simulink model "asbCubeSatVisualization"  (R2025b)
settings: configuration reference "CubeSatConfigSet" (kept outside this file)
StopFcn:
  | exSatScenMdl = bdroot(gcs);
  | exSatScenBlk = exSatScenMdl + "/Satellite Scenario Playback";
  | 
  | % If workspace blocks are stored in single output variable, need to access from there
  | if get_param(exSatScenMdl, "ReturnWorkspaceOutputs") == "on"
  |     exSatScenOutVar = get_param(exSatScenMdl, "ReturnWorkspaceOutputsName");
  |     if exist(exSatScenOutVar, "var")
  |         exSatScenTimeData = eval(exSatScenOutVar).exSatScenTimeData;
  |         exSatScenPositionData = eval(exSatScenOutVar).exSatScenPositionData;
  |         exSatScenVelocityData = eval(exSatScenOutVar).exSatScenVelocityData;
  |         exSatScenAttitudeData = eval(exSatScenOutVar).exSatScenAttitudeData;
  |     end
  | end
  | 
  | % If variables exist, create scenario (variables are not created if called with sim command)
  | if exist("exSatScenTimeData", "var") && exist("exSatScenPositionData", "var") && exist("exSatScenVelocityData", "var") && exist("exSatScenAttitudeData", "var")
  |     % Create satellite scenario from variables accessed above or directly from workspace
  |     exSatScenario = Aero.spacecraft.analysis.createSatelliteScenarioFromSim(exSatScenBlk, ...
  |         exSatScenTimeData, exSatScenPositionData, exSatScenVelocityData, exSatScenAttitudeData);
  | end
  | 
  | clear exSatScenBlk exSatScenMdl exSatScenOutVar exSatScenTimeData exSatScenPositionData exSatScenVelocityData exSatScenAttitudeData
libraries: simulink x12
settings Model: DataDictionary=asbCubeSatArchInterfaceData.sldd  Creator=The MathWorks, Inc.  LastModifiedBy=The MathWorks, Inc.
settings ConfigSetRef: SourceName=CubeSatConfigSet

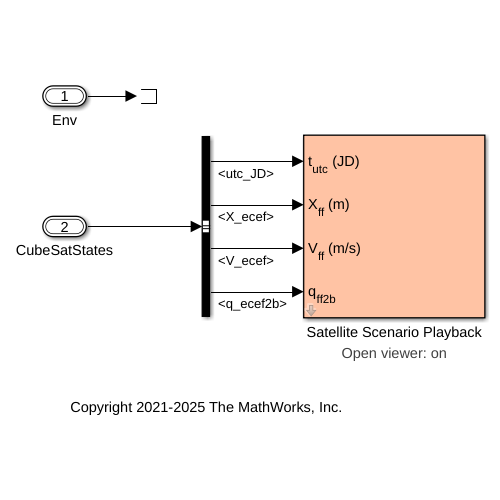
[thumbnail: Simulink's stored preview of the top-level diagram]
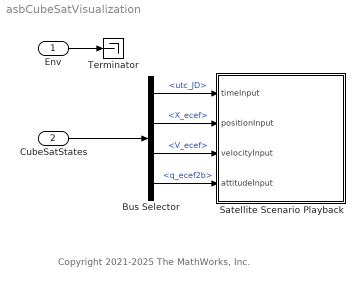
== system asbCubeSatVisualization ==
  note: Copyright 2021-2025 The MathWorks, Inc.
  Env : Inport  OutDataTypeStr=Bus: EnvBus
  CubeSatStates : Inport  Port=2  OutDataTypeStr=Bus: StatesOutBus
  Bus Selector : BusSelector  OutputSignals=utc_JD,X_ecef,V_ecef,q_ecef2b
  Satellite Scenario Playback : Subsystem  mask{openViewer=on, stateFrame=ECEF (Fixed-frame), useVelocity=on, useAttitude=on, attitudeFrame=ECEF (Fixed-frame), satName=Satellite, showTriad=on, show3dModel=on, showFOV=on, fovHalfAngle=30, scenarioStep=60}
      mask prompts: openViewer "Enable Satellite Scenario Viewer playback animation"; stateFrame "State coordinate frame:"; useVelocity "Add velocity port"; useAttitude "Add attitude port"; attitudeFrame "Attitude coordinate frame (Frame to Body):"; satName "Satellite or constellation label:"; showTriad "Show coordinate axis triad (Body frame)"; show3dModel "Show 3D satellite model"; showFOV "Add sensor field-of-view (FOV)"; fovHalfAngle "FOV half angle (deg):"; scenarioStep "Satellite scenario sample time (s):"
      mask init:
      | ports = Aero.spacecraft.analysis.satelliteScenarioPlaybackMaskCallback(gcb, "init");
      settings: AttributesFormatString=Open viewer: %<openViewer>
      mask Callback openViewer: Aero.spacecraft.analysis.satelliteScenarioPlaybackMaskCallback(gcb, "viewer");
      mask TypeOptions stateFrame: Inertial (ICRF) | ECEF (Fixed-frame) | Geographic
      mask Callback useAttitude: Aero.spacecraft.analysis.satelliteScenarioPlaybackMaskCallback(gcb, "attitude");
      mask TypeOptions attitudeFrame: Inertial (ICRF) | ECEF (Fixed-frame) | NED
      mask Callback showFOV: Aero.spacecraft.analysis.satelliteScenarioPlaybackMaskCallback(gcb, "fov");
      mask DialogControl DescGroupVar Prompt: Satellite Scenario Viewer Playback Animation
      mask DialogControl DescTextVar Prompt: <html><p>Create a satellite scenario object and launch the Satellite Scenario Viewer using the trajectories provided as inputs to the block.</p><p>If playback animation is enabled, the block opens Satellite Scenario Viewer after the model simulation has stopped. The viewer will not launch if the model is run using the <tt>sim</tt> command.</p> <p>To add additional satellites, ground stations, or platforms to the scenario and perform mission analysis, including line-of-sight access and eclipse analysis, use the base workspace variable <tt>exSatScenario</tt>.</p></html>
      mask DialogControl Container3 Prompt: Parameters
      mask DialogControl Container4 Prompt: Trajectory
      mask DialogControl ParameterGroupVar Prompt: Playback
      mask DialogControl SatelliteScenarioPlaybackTag Prompt: SatelliteScenarioPlaybackTag
      mask Display:
      | port_label(ports(1).type,ports(1).port,ports(1).txt,'texmode','on');
      | port_label(ports(2).type,ports(2).port,ports(2).txt,'texmode','on');
      | port_label(ports(3).type,ports(3).port,ports(3).txt,'texmode','on');
      | port_label(ports(4).type,ports(4).port,ports(4).txt,'texmode','on');
  Terminator : Terminator
  wires:
  CubeSatStates/1 -> Bus Selector/1
  Env/1 -> Terminator/1
  Bus Selector/4 -> Satellite Scenario Playback/4(attitudeInput)  "<q_ecef2b>"
  Bus Selector/3 -> Satellite Scenario Playback/3(velocityInput)  "<V_ecef>"
  Bus Selector/2 -> Satellite Scenario Playback/2(positionInput)  "<X_ecef>"
  Bus Selector/1 -> Satellite Scenario Playback/1(timeInput)  "<utc_JD>"

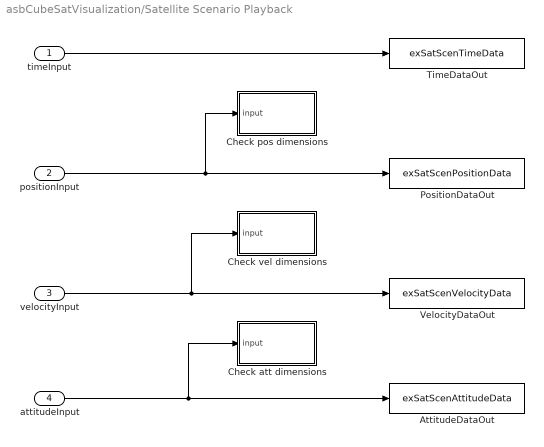
== system asbCubeSatVisualization/Satellite Scenario Playback ==
  timeInput : Inport  PortDimensions=1
  positionInput : Inport  Port=2  Unit=m
  velocityInput : Inport  Port=3  Unit=m/s
  attitudeInput : Inport  Port=4
  AttitudeDataOut : ToWorkspace  VariableName=exSatScenAttitudeData  SampleTime=-1
  Check att dimensions : Subsystem  mask{N=4, AssertionFailFcn=error("Attitude input must be be a vector with 4 elements or a 2-D array of size [m x 4].")}
      mask prompts: N "State dimension (N):"; AssertionFailFcn "Simulink:blkprm_prompts:AssertionCallback"
      mask TypeOptions AssertionFailFcn: Assertion/AssertionFailFcn | Second check/Assertion/AssertionFailFcn
      mask DialogControl DescGroupVar Prompt: Assert expected dimensions
      mask DialogControl DescTextVar Prompt: Assert that input signal is size N or size M x N where M is the number of satellites. N is 3 for position and velocity, and 4 for attitude (quaternions).
      mask DialogControl AssertionFailFcn Prompt: Simulation callback when assertion fails:
  Check pos dimensions : Subsystem  mask{N=3, AssertionFailFcn=error("Position input must be be a vector with 3 elements or a 2-D array of size [m x 3].")}
      mask prompts: N "State dimension (N):"; AssertionFailFcn "Simulink:blkprm_prompts:AssertionCallback"
      mask TypeOptions AssertionFailFcn: Assertion/AssertionFailFcn | Second check/Assertion/AssertionFailFcn
      mask DialogControl DescGroupVar Prompt: Assert expected dimensions
      mask DialogControl DescTextVar Prompt: Assert that input signal is size N or size M x N where M is the number of satellites. N is 3 for position and velocity, and 4 for attitude (quaternions).
      mask DialogControl AssertionFailFcn Prompt: Simulation callback when assertion fails:
  Check vel dimensions : Subsystem  mask{N=3, AssertionFailFcn=error("Velocity input must be be a vector with 3 elements or a 2-D array of size [m x 3].")}
      mask prompts: N "State dimension (N):"; AssertionFailFcn "Simulink:blkprm_prompts:AssertionCallback"
      mask TypeOptions AssertionFailFcn: Assertion/AssertionFailFcn | Second check/Assertion/AssertionFailFcn
      mask DialogControl DescGroupVar Prompt: Assert expected dimensions
      mask DialogControl DescTextVar Prompt: Assert that input signal is size N or size M x N where M is the number of satellites. N is 3 for position and velocity, and 4 for attitude (quaternions).
      mask DialogControl AssertionFailFcn Prompt: Simulation callback when assertion fails:
  PositionDataOut : ToWorkspace  VariableName=exSatScenPositionData  SampleTime=-1
  TimeDataOut : ToWorkspace  VariableName=exSatScenTimeData  SampleTime=-1
  VelocityDataOut : ToWorkspace  VariableName=exSatScenVelocityData  SampleTime=-1
  wires:
  positionInput/1 -> PositionDataOut/1, Check pos dimensions/1(input)
  velocityInput/1 -> Check vel dimensions/1(input), VelocityDataOut/1
  attitudeInput/1 -> Check att dimensions/1(input), AttitudeDataOut/1
  timeInput/1 -> TimeDataOut/1

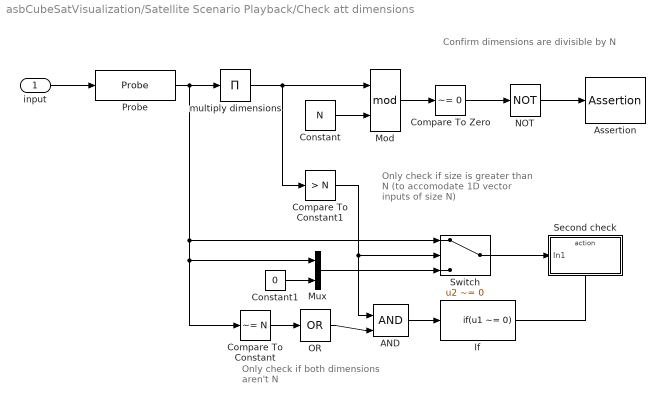
== system asbCubeSatVisualization/Satellite Scenario Playback/Check att dimensions ==
  note: Only check if both dimensions aren't N
  note: Only check if size is greater than N (to accomodate 1D vector inputs of size N)
  note: Confirm dimensions are divisible by N
  input : Inport
  AND : Logic  IconShape=distinctive  AllPortsSameDT=off  OutDataTypeStr=boolean
  Assertion : Assertion  AssertionFailFcn="error(\"Attitude input must be be a vector with 4 elements or a 2-D array of size [m x 4].\")"
  Compare To Constant : simulink/Logic and Bit Operations/Compare To Constant  relop=~=  const=N  OutDataTypeStr=boolean  ZeroCross=off
  Compare To Constant1 : simulink/Logic and Bit Operations/Compare To Constant  relop=>  const=N  OutDataTypeStr=boolean  ZeroCross=off
  Compare To Zero : simulink/Logic and Bit Operations/Compare To Zero  relop=~=  OutDataTypeStr=boolean  ZeroCross=off
  Constant : Constant  Value=N  OutDataTypeStr=uint8
  Constant1 : Constant  Value=0  OutDataTypeStr=uint8
  If : If  IfExpression=u1 ~= 0  ShowElse=off  ZeroCross=off
  Mod : Math  Operator=mod
  Mux : Mux  Inputs=2
  NOT : Logic  Operator=NOT  IconShape=distinctive  AllPortsSameDT=off  OutDataTypeStr=boolean
  OR : Logic  Operator=OR  Inputs=1  IconShape=distinctive  AllPortsSameDT=off  OutDataTypeStr=boolean
  Probe : Probe  ProbeWidth=off  ProbeSampleTime=off  ProbeComplexSignal=off  ProbeSignalDimensions=on  ProbeDimensionsDataType=uint8
  Second check : Subsystem  TreatAsAtomicUnit=on
  Switch : Switch  Criteria=u2 ~= 0  SaturateOnIntegerOverflow=off  InputSameDT=off
  multiply dimensions : Product  Inputs=*  OutDataTypeStr=uint8
  wires:
  input/1 -> Probe/1
  Constant/1 -> Mod/2
  Compare To Zero/1 -> NOT/1
  Mod/1 -> Compare To Zero/1
  NOT/1 -> Assertion/1
  multiply dimensions/1 -> Compare To Constant1/1, Mod/1
  Probe/1 -> Mux/1, Compare To Constant/1, Switch/1, multiply dimensions/1
  Compare To Constant/1 -> OR/1
  OR/1 -> AND/2
  If/1 -> Second check/Action
  Compare To Constant1/1 -> Switch/2, AND/1
  AND/1 -> If/1
  Constant1/1 -> Mux/2
  Mux/1 -> Switch/3
  Switch/1 -> Second check/1(In1)

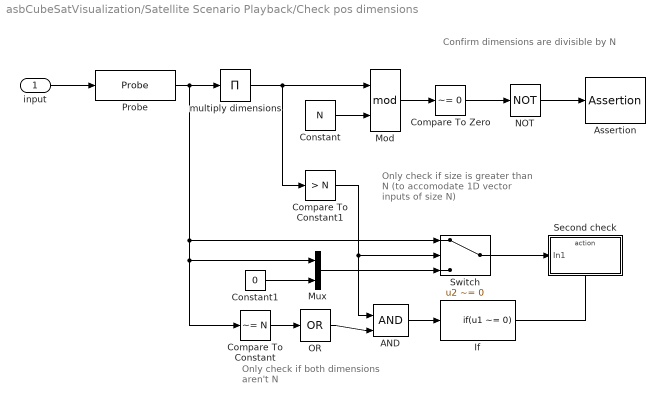
== system asbCubeSatVisualization/Satellite Scenario Playback/Check pos dimensions ==
  note: Only check if both dimensions aren't N
  note: Only check if size is greater than N (to accomodate 1D vector inputs of size N)
  note: Confirm dimensions are divisible by N
  input : Inport
  AND : Logic  IconShape=distinctive  AllPortsSameDT=off  OutDataTypeStr=boolean
  Assertion : Assertion  AssertionFailFcn="error(\"Position input must be be a vector with 3 elements or a 2-D array of size [m x 3].\")"
  Compare To Constant : simulink/Logic and Bit Operations/Compare To Constant  relop=~=  const=N  OutDataTypeStr=boolean  ZeroCross=off
  Compare To Constant1 : simulink/Logic and Bit Operations/Compare To Constant  relop=>  const=N  OutDataTypeStr=boolean  ZeroCross=off
  Compare To Zero : simulink/Logic and Bit Operations/Compare To Zero  relop=~=  OutDataTypeStr=boolean  ZeroCross=off
  Constant : Constant  Value=N  OutDataTypeStr=uint8
  Constant1 : Constant  Value=0  OutDataTypeStr=uint8
  If : If  IfExpression=u1 ~= 0  ShowElse=off  ZeroCross=off
  Mod : Math  Operator=mod
  Mux : Mux  Inputs=2
  NOT : Logic  Operator=NOT  IconShape=distinctive  AllPortsSameDT=off  OutDataTypeStr=boolean
  OR : Logic  Operator=OR  Inputs=1  IconShape=distinctive  AllPortsSameDT=off  OutDataTypeStr=boolean
  Probe : Probe  ProbeWidth=off  ProbeSampleTime=off  ProbeComplexSignal=off  ProbeSignalDimensions=on  ProbeDimensionsDataType=uint8
  Second check : Subsystem  TreatAsAtomicUnit=on
  Switch : Switch  Criteria=u2 ~= 0  SaturateOnIntegerOverflow=off  InputSameDT=off
  multiply dimensions : Product  Inputs=*  OutDataTypeStr=uint8
  wires:
  input/1 -> Probe/1
  Constant/1 -> Mod/2
  Compare To Zero/1 -> NOT/1
  Mod/1 -> Compare To Zero/1
  NOT/1 -> Assertion/1
  multiply dimensions/1 -> Compare To Constant1/1, Mod/1
  Probe/1 -> Mux/1, Compare To Constant/1, Switch/1, multiply dimensions/1
  Compare To Constant/1 -> OR/1
  OR/1 -> AND/2
  If/1 -> Second check/Action
  Compare To Constant1/1 -> Switch/2, AND/1
  AND/1 -> If/1
  Constant1/1 -> Mux/2
  Mux/1 -> Switch/3
  Switch/1 -> Second check/1(In1)

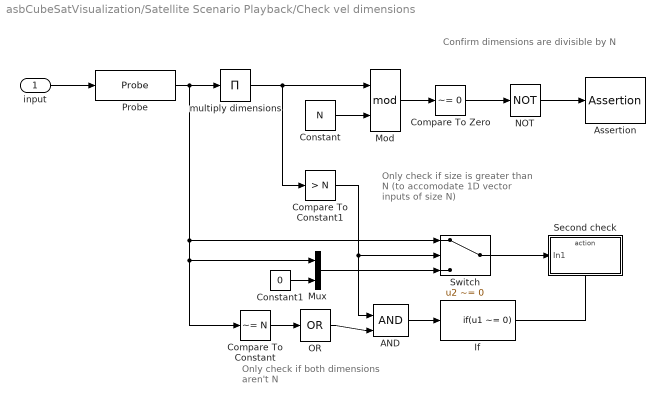
== system asbCubeSatVisualization/Satellite Scenario Playback/Check vel dimensions ==
  note: Confirm dimensions are divisible by N
  note: Only check if size is greater than N (to accomodate 1D vector inputs of size N)
  note: Only check if both dimensions aren't N
  input : Inport
  AND : Logic  IconShape=distinctive  AllPortsSameDT=off  OutDataTypeStr=boolean
  Assertion : Assertion  AssertionFailFcn="error(\"Velocity input must be be a vector with 3 elements or a 2-D array of size [m x 3].\")"
  Compare To Constant : simulink/Logic and Bit Operations/Compare To Constant  relop=~=  const=N  OutDataTypeStr=boolean  ZeroCross=off
  Compare To Constant1 : simulink/Logic and Bit Operations/Compare To Constant  relop=>  const=N  OutDataTypeStr=boolean  ZeroCross=off
  Compare To Zero : simulink/Logic and Bit Operations/Compare To Zero  relop=~=  OutDataTypeStr=boolean  ZeroCross=off
  Constant : Constant  Value=N  OutDataTypeStr=uint8
  Constant1 : Constant  Value=0  OutDataTypeStr=uint8
  If : If  IfExpression=u1 ~= 0  ShowElse=off  ZeroCross=off
  Mod : Math  Operator=mod
  Mux : Mux  Inputs=2
  NOT : Logic  Operator=NOT  IconShape=distinctive  AllPortsSameDT=off  OutDataTypeStr=boolean
  OR : Logic  Operator=OR  Inputs=1  IconShape=distinctive  AllPortsSameDT=off  OutDataTypeStr=boolean
  Probe : Probe  ProbeWidth=off  ProbeSampleTime=off  ProbeComplexSignal=off  ProbeSignalDimensions=on  ProbeDimensionsDataType=uint8
  Second check : Subsystem  TreatAsAtomicUnit=on
  Switch : Switch  Criteria=u2 ~= 0  SaturateOnIntegerOverflow=off  InputSameDT=off
  multiply dimensions : Product  Inputs=*  OutDataTypeStr=uint8
  wires:
  Switch/1 -> Second check/1(In1)
  Mux/1 -> Switch/3
  Constant1/1 -> Mux/2
  AND/1 -> If/1
  Compare To Constant1/1 -> AND/1, Switch/2
  If/1 -> Second check/Action
  OR/1 -> AND/2
  Compare To Constant/1 -> OR/1
  Probe/1 -> multiply dimensions/1, Switch/1, Compare To Constant/1, Mux/1
  multiply dimensions/1 -> Mod/1, Compare To Constant1/1
  NOT/1 -> Assertion/1
  Mod/1 -> Compare To Zero/1
  Compare To Zero/1 -> NOT/1
  Constant/1 -> Mod/2
  input/1 -> Probe/1

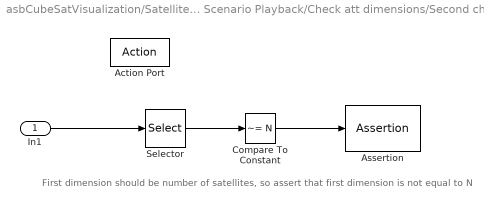
== system asbCubeSatVisualization/Satellite Scenario Playback/Check att dimensions/Second check ==
  note: First dimension should be number of satellites, so assert that first dimension is not equal to N
  In1 : Inport
  Action Port : ActionPort  ActionPortLabel=if(u1 ~= 0)
  Assertion : Assertion  AssertionFailFcn="error(\"Attitude input must be be a vector with 4 elements or a 2-D array of size [m x 4].\")"
  Compare To Constant : simulink/Logic and Bit Operations/Compare To Constant  relop=~=  const=N  OutDataTypeStr=boolean  ZeroCross=off
  Selector : Selector  InputPortWidth=2  IndexOptions=Index vector (dialog)  Indices=[1]  OutputSizes=1
  wires:
  Selector/1 -> Compare To Constant/1
  In1/1 -> Selector/1
  Compare To Constant/1 -> Assertion/1

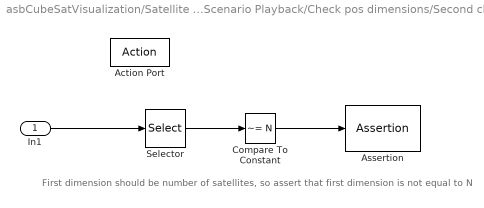
== system asbCubeSatVisualization/Satellite Scenario Playback/Check pos dimensions/Second check ==
  note: First dimension should be number of satellites, so assert that first dimension is not equal to N
  In1 : Inport
  Action Port : ActionPort  ActionPortLabel=if(u1 ~= 0)
  Assertion : Assertion  AssertionFailFcn="error(\"Position input must be be a vector with 3 elements or a 2-D array of size [m x 3].\")"
  Compare To Constant : simulink/Logic and Bit Operations/Compare To Constant  relop=~=  const=N  OutDataTypeStr=boolean  ZeroCross=off
  Selector : Selector  InputPortWidth=2  IndexOptions=Index vector (dialog)  Indices=[1]  OutputSizes=1
  wires:
  Selector/1 -> Compare To Constant/1
  In1/1 -> Selector/1
  Compare To Constant/1 -> Assertion/1

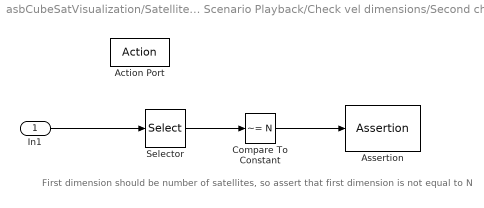
== system asbCubeSatVisualization/Satellite Scenario Playback/Check vel dimensions/Second check ==
  note: First dimension should be number of satellites, so assert that first dimension is not equal to N
  In1 : Inport
  Action Port : ActionPort  ActionPortLabel=if(u1 ~= 0)
  Assertion : Assertion  AssertionFailFcn="error(\"Velocity input must be be a vector with 3 elements or a 2-D array of size [m x 3].\")"
  Compare To Constant : simulink/Logic and Bit Operations/Compare To Constant  relop=~=  const=N  OutDataTypeStr=boolean  ZeroCross=off
  Selector : Selector  InputPortWidth=2  IndexOptions=Index vector (dialog)  Indices=[1]  OutputSizes=1
  wires:
  Compare To Constant/1 -> Assertion/1
  In1/1 -> Selector/1
  Selector/1 -> Compare To Constant/1
